simulink model "lab2_var9"  (R2023b)
settings: Solver=VariableStepAuto  StartTime=0.0  StopTime=10  RelTol=1e-3
settings Model: Creator=Эмма  LastModifiedBy=Эмма

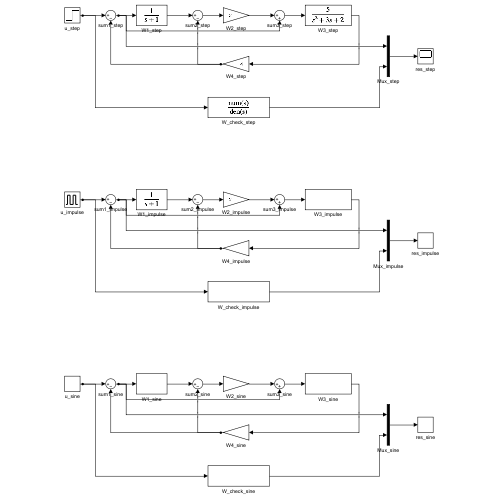
[thumbnail: Simulink's stored preview of the top-level diagram]
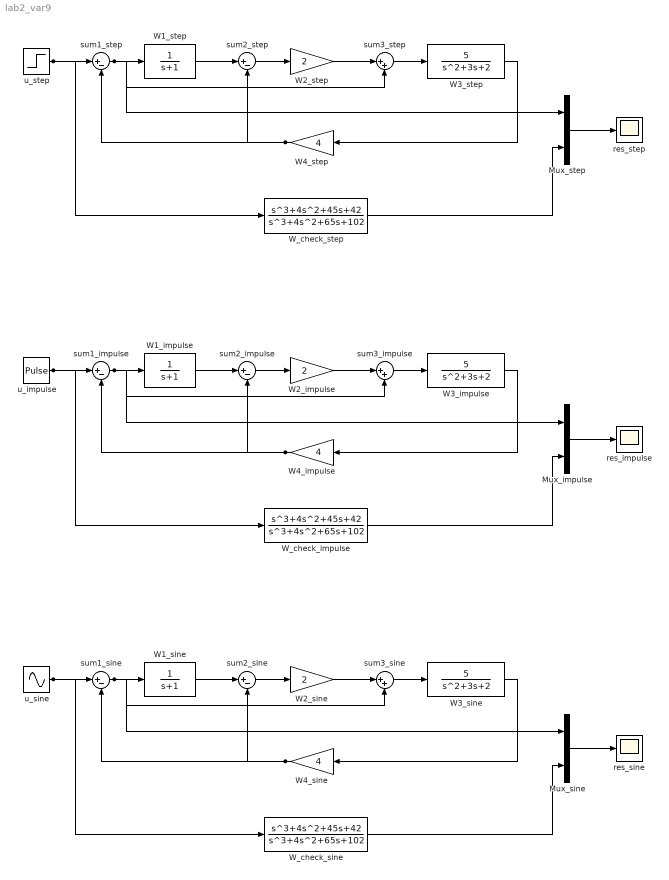
== system lab2_var9 ==
  Mux_impulse : Mux  Inputs=2
  Mux_sine : Mux  Inputs=2
  Mux_step : Mux  Inputs=2
  W1_impulse : TransferFcn  Denominator=[1 1]
  W1_sine : TransferFcn  Denominator=[1 1]
  W1_step : TransferFcn  Denominator=[1 1]
  W2_impulse : Gain  Gain=2
  W2_sine : Gain  Gain=2
  W2_step : Gain  Gain=2
  W3_impulse : TransferFcn  Numerator=[5]  Denominator=[1 3 2]
  W3_sine : TransferFcn  Numerator=[5]  Denominator=[1 3 2]
  W3_step : TransferFcn  Numerator=[5]  Denominator=[1 3 2]
  W4_impulse : Gain  Gain=4
  W4_sine : Gain  Gain=4
  W4_step : Gain  Gain=4
  W_check_impulse : TransferFcn  Numerator=[1 4 45 42]  Denominator=[1 4 65 102]
  W_check_sine : TransferFcn  Numerator=[1 4 45 42]  Denominator=[1 4 65 102]
  W_check_step : TransferFcn  Numerator=[1 4 45 42]  Denominator=[1 4 65 102]
  res_impulse : Scope
  res_sine : Scope
  res_step : Scope
  sum1_impulse : Sum  Inputs=|+-
  sum1_sine : Sum  Inputs=|+-
  sum1_step : Sum  Inputs=|+-
  sum2_impulse : Sum  Inputs=|+-
  sum2_sine : Sum  Inputs=|+-
  sum2_step : Sum  Inputs=|+-
  sum3_impulse : Sum  Inputs=|++
  sum3_sine : Sum  Inputs=|++
  sum3_step : Sum  Inputs=|++
  u_impulse : DiscretePulseGenerator  PulseType=Time based  Period=10  PulseWidth=5
  u_sine : Sin  SampleTime=0
  u_step : Step  SampleTime=0
  wires:
  u_step/1 -> sum1_step/1, W_check_step/1
  sum1_step/1 -> W1_step/1, sum3_step/2, Mux_step/1
  W1_step/1 -> sum2_step/1
  sum2_step/1 -> W2_step/1
  W2_step/1 -> sum3_step/1
  sum3_step/1 -> W3_step/1
  W3_step/1 -> W4_step/1
  W4_step/1 -> sum1_step/2, sum2_step/2
  W_check_step/1 -> Mux_step/2
  Mux_step/1 -> res_step/1
  u_impulse/1 -> sum1_impulse/1, W_check_impulse/1
  sum1_impulse/1 -> W1_impulse/1, sum3_impulse/2, Mux_impulse/1
  W1_impulse/1 -> sum2_impulse/1
  sum2_impulse/1 -> W2_impulse/1
  W2_impulse/1 -> sum3_impulse/1
  sum3_impulse/1 -> W3_impulse/1
  W3_impulse/1 -> W4_impulse/1
  W4_impulse/1 -> sum1_impulse/2, sum2_impulse/2
  W_check_impulse/1 -> Mux_impulse/2
  Mux_impulse/1 -> res_impulse/1
  u_sine/1 -> sum1_sine/1, W_check_sine/1
  sum1_sine/1 -> W1_sine/1, sum3_sine/2, Mux_sine/1
  W1_sine/1 -> sum2_sine/1
  sum2_sine/1 -> W2_sine/1
  W2_sine/1 -> sum3_sine/1
  sum3_sine/1 -> W3_sine/1
  W3_sine/1 -> W4_sine/1
  W4_sine/1 -> sum1_sine/2, sum2_sine/2
  W_check_sine/1 -> Mux_sine/2
  Mux_sine/1 -> res_sine/1
